simulink model "mppt"  (R2023b)
settings: Solver=VariableStepAuto  StartTime=0.0  StopTime=3.0  RelTol=1e-3
libraries: spsSeriesRLCBranchLib x4, spsCurrentMeasurementLib x1, spsDiodeLib x1, spsIGBTLib x1, spsPVArrayLib x1, eePwmGenerator x1, spsStairGeneratorLib x1, spsVoltageMeasurementLib x1, sps_lib x1
settings Model: Creator=ACER  LastModifiedBy=ACER

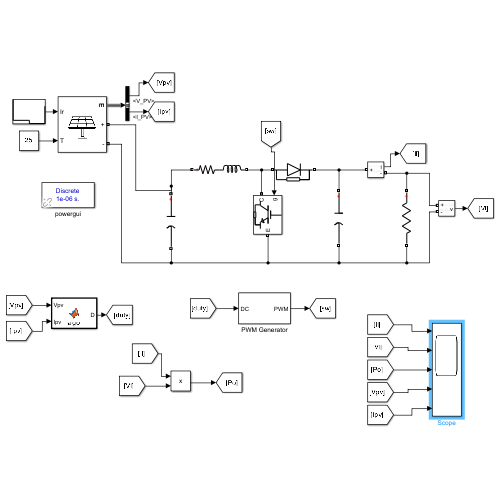
[thumbnail: Simulink's stored preview of the top-level diagram]
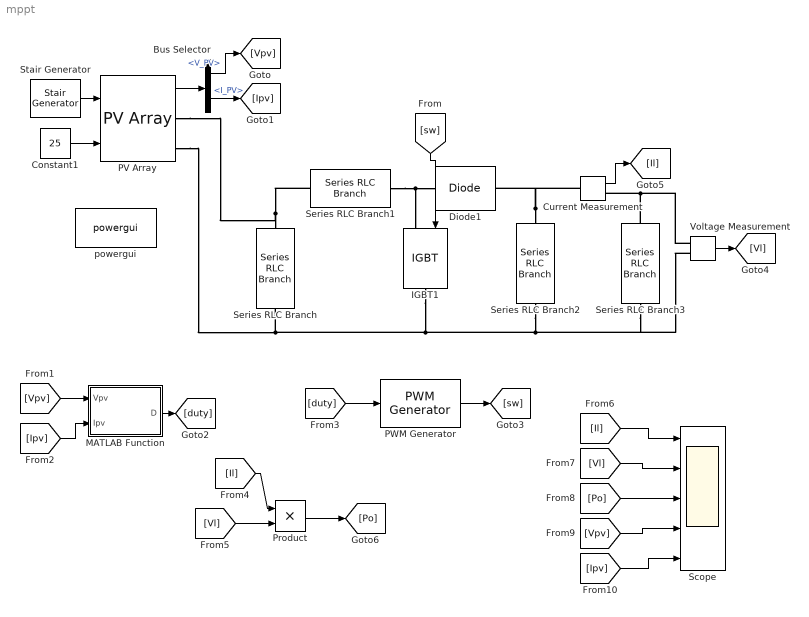
== system mppt ==
  Bus Selector : BusSelector  OutputSignals=V_PV,I_PV
  Constant1 : Constant  Value=25
  Current Measurement : spsCurrentMeasurementLib/Current Measurement  PhasorSimulation=off  OutputType=Complex  PSBequivalent=0
  Diode1 : spsDiodeLib/Diode  Ron=0.001  Lon=0  Vf=0.8  IC=0  UseSnubber=0  Rs=500  Cs=250e-9  Measurements=off
  IGBT1 : spsIGBTLib/IGBT  Ron=0.001  Lon=0  Vf=1  Tf=1e-6  Tt=2e-6  IC=0  Rs=1e5  Cs=inf  Measurements=off
  MATLAB Function : MATLAB Function  TreatAsAtomicUnit=on
  PV Array : spsPVArrayLib/PV Array  Npar=1  Nser=3  PlotType=array @ 1000 W/m2 & specified temperatures  S_vec="[ 1000  500  100 ]"  Temp_C_vec="[ 45 25  ]"  ModuleName=SunPower SPR-400E-WHT-D  PlotWhenSelected=off  Pm=400.221  Ncell=128  Voc=85.3  Isc=5.87  Vm=72.9  Im=5.49  beta_Voc_pc=-0.229  alpha_Isc_pc=0.030698  beta_Voc=-0.19534  alpha_Isc=0.001802  IL=5.8772  I0=6.9148e-13  nI=0.87221  Rsh=451.8291  Rs=0.55721  RobustModel=off  RobustCellTemperature=313.3991  BAL=on  Tc=1e-6  Tfilter=5e-5
  PWM Generator : eePwmGenerator/PWM Generator  CarrCount=Up  Tper=0.001  Tdelay=0  Ts=5e-5
  Product : Product
  Scope : Scope  NumInputPorts=5
  Series RLC Branch : spsSeriesRLCBranchLib/Series RLC Branch  LConnTagsString=__new0  RConnTagsString=__new0  BranchType=C  Resistance=1  Inductance=1e-3  SetiL0=off  InitialCurrent=0  Capacitance=100e-6  Setx0=off  InitialVoltage=0  Measurements=None
  Series RLC Branch1 : spsSeriesRLCBranchLib/Series RLC Branch  LConnTagsString=__new0  RConnTagsString=__new0  BranchType=RL  Resistance=.1  Inductance=5e-3  SetiL0=off  InitialCurrent=0  Capacitance=1e-6  Setx0=off  InitialVoltage=0  Measurements=None
  Series RLC Branch2 : spsSeriesRLCBranchLib/Series RLC Branch  LConnTagsString=__new0  RConnTagsString=__new0  BranchType=C  Resistance=1  Inductance=1e-3  SetiL0=off  InitialCurrent=0  Capacitance=3300e-6  Setx0=off  InitialVoltage=0  Measurements=None
  Series RLC Branch3 : spsSeriesRLCBranchLib/Series RLC Branch  LConnTagsString=__new0  RConnTagsString=__new0  BranchType=R  Resistance=10  Inductance=1e-3  SetiL0=off  InitialCurrent=0  Capacitance=1e-6  Setx0=off  InitialVoltage=0  Measurements=None
  Stair Generator : spsStairGeneratorLib/Stair Generator  t=[0, .5, 1.5, 2.5]  e=[1000, 350, 250, 800]  Ts=0
  Voltage Measurement : spsVoltageMeasurementLib/Voltage Measurement  PhasorSimulation=off  OutputType=Complex  PSBequivalent=0
  powergui : sps_lib/powergui  Priority=1  SimulationMode=Discrete  SampleTime=1e-6  frequency=60  Iterations=50  frequencyindice=0  Pbase=100e6  ErrMax=1e-4  UnitsV=kV  UnitsW=MW  buscounter=0  FunctionMessages=off  echomessages=off  EnableUseOfTLC=off  CurrentSourceSwitches=off  DisableSnubberDevices=off  DisableRonSwitches=off  DisableVfSwitches=off  DisplayEquations=off  AutomaticDiscreteSolvers=off  SolverType=Tustin/Backward Euler (TBE)  Interpol=off  ExternalGateDelay=off  methode=off  Ts=100  x0status=blocks  SPID=on  SwTol=0  HookPort=off  NonlinearTolerance=1e-4  nMaxIteration=100  ContinueOnMaxIteration=off  RestoreLinks=warning  ResistiveCurrentMeasurement=off  Frange=[0:2:500]  Ylog=off  Xlog=on  ShowGrid=off  save=off  variable=ZData  structure=0  ZoomFFT=off  StartTime=0.0  cycles=1  DisplayStyle=1  fundamental=60  FreqAxis=off  MaxFrequency=1000  frequencyindicesteady=1  RmsSteady=1  display=off
  wires:
  Stair Generator/1 -> PV Array/1
  Constant1/1 -> PV Array/2
  PV Array/1 -> Bus Selector/1
  Bus Selector/1 -> [Vpv]  "<V_PV>"
  Bus Selector/2 -> [Ipv]  "<I_PV>"
  MATLAB Function/1(D) -> [duty]
  [sw] -> IGBT1/1
  [Vpv] -> MATLAB Function/1(Vpv)
  [Ipv] -> MATLAB Function/2(Ipv)
  [duty] -> PWM Generator/1
  PWM Generator/1 -> [sw]
  Voltage Measurement/1 -> [Vl]
  Current Measurement/1 -> [Il]
  [Il] -> Product/1
  [Vl] -> Product/2
  Product/1 -> [Po]
  [Il] -> Scope/1
  [Vl] -> Scope/2
  [Po] -> Scope/3
  [Vpv] -> Scope/4
  [Ipv] -> Scope/5
  connections:
  PV Array/RConn1 -- Series RLC Branch1/LConn1 -- Series RLC Branch/LConn1
  Series RLC Branch2/LConn1 -- Current Measurement/LConn1 -- Diode1/RConn1
  PV Array/RConn2 -- Voltage Measurement/LConn2 -- Series RLC Branch3/RConn1 -- Series RLC Branch2/RConn1 -- IGBT1/RConn1 -- Series RLC Branch/RConn1
  Series RLC Branch1/RConn1 -- IGBT1/LConn1 -- Diode1/LConn1
  Series RLC Branch3/LConn1 -- Voltage Measurement/LConn1 -- Current Measurement/RConn1

== matlab function mppt/MATLAB Function ==
  data: Vpv input; D output; Ipv input
function D = algo(Vpv, Ipv)

persistent Dprev Pprev Vprev

if isempty(Dprev)
    Dprev = .7;
    Pprev = 190;
    Vprev = 2000;
end

delD = 125e-6;

Ppv = Vpv * Ipv;

if (Ppv - Pprev) ~= 0
    if (Ppv - Pprev) > 0
        if (Vpv - Vprev) > 0
            D = Dprev - delD;
        else 
            D = Dprev + delD;
        end
    else
        if (Vpv - Vprev) > 0
            D = Dprev + delD;
        else 
            D = Dprev - delD;
        end
    end
else
    D = Dprev;
end

Dprev = D;
Vprev = Vpv;
Pprev = Ppv;
